simulink model "dq_current_controller_discrete"  (R2025b)
settings: Solver=FixedStepDiscrete  FixedStep=control.currentLoopPeriod_s
undefined symbols (not defined in the file): control, DiscIntNeverNeededParam, motor
settings Model: Creator=semih  LastModifiedBy=Semih
settings SFSimCC: SimGPUStackLimitPerThread=51200  SimGPUMallocThreshold=200
settings RTWCC: GPUStackLimitPerThread=51200  GPUMallocThreshold=200
settings GRTTargetCC: CombineOutputUpdateFcns=off

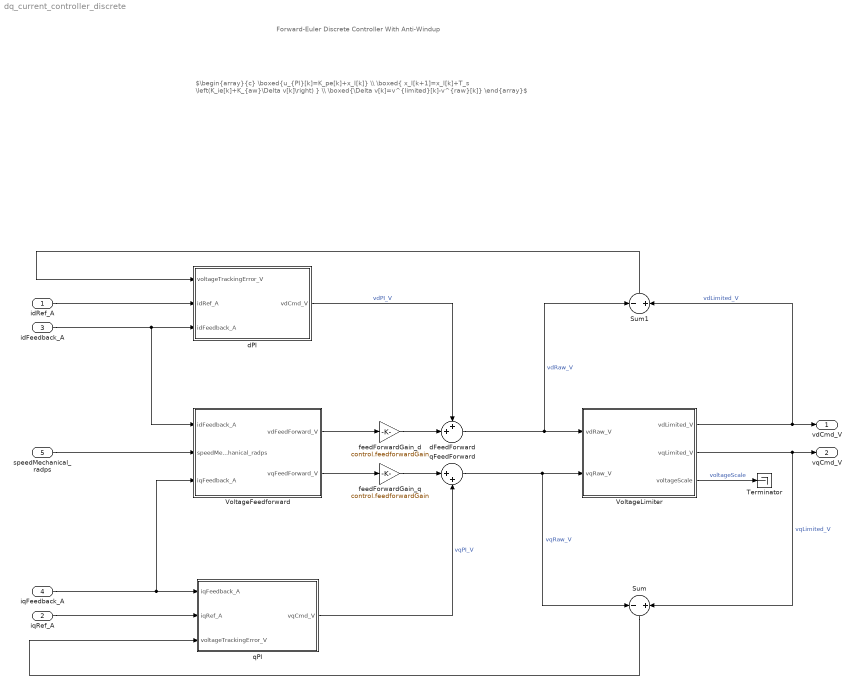
== system dq_current_controller_discrete ==
  note: $\begin{array}{c} \boxed{u_{PI}[k]=K_pe[k]+x_I[k]} \\ \boxed{ x_I[k+1]=x_I[k]+T_s \left(K_ie[k]+K_{aw}\Delta v[k]\right) } \\ \boxed{\Delta v[k]=v^{limited}[k]-v^{raw}[k]} \end{array}$
  note: Forward-Euler Discrete Controller
      | With Anti-Windup
  idRef_A : Inport
  iqRef_A : Inport  Port=2
  idFeedback_A : Inport  Port=3
  iqFeedback_A : Inport  Port=4
  speedMechanical_radps : Inport  Port=5
  Sum : Sum  Inputs=-+
  Sum1 : Sum  Inputs=-+
  Terminator : Terminator
  VoltageFeedforward : Subsystem
  VoltageLimiter : Subsystem
  dFeedForward : Sum  Inputs=++|
  dPI : Subsystem
  feedForwardGain_d : Gain  Gain=control.feedforwardGain
  feedForwardGain_q : Gain  Gain=control.feedforwardGain
  qFeedForward : Sum  Inputs=|++
  qPI : Subsystem
  vdCmd_V : Outport
  vqCmd_V : Outport  Port=2
  wires:
  dPI/1(vdCmd_V) -> dFeedForward/1  "vdPI_V"
  qPI/1(vqCmd_V) -> qFeedForward/2  "vqPI_V"
  VoltageFeedforward/2(vqFeedForward_V) -> feedForwardGain_q/1
  VoltageFeedforward/1(vdFeedForward_V) -> feedForwardGain_d/1
  feedForwardGain_q/1 -> qFeedForward/1
  feedForwardGain_d/1 -> dFeedForward/2
  idRef_A/1 -> dPI/2(idRef_A)
  idFeedback_A/1 -> VoltageFeedforward/1(idFeedback_A), dPI/3(idFeedback_A)
  speedMechanical_radps/1 -> VoltageFeedforward/2(speedMechanical_radps)
  iqFeedback_A/1 -> qPI/1(iqFeedback_A), VoltageFeedforward/3(iqFeedback_A)
  dFeedForward/1 -> Sum1/1, VoltageLimiter/1(vdRaw_V)  "vdRaw_V"
  qFeedForward/1 -> Sum/1, VoltageLimiter/2(vqRaw_V)  "vqRaw_V"
  VoltageLimiter/1(vdLimited_V) -> Sum1/2, vdCmd_V/1  "vdLimited_V"
  VoltageLimiter/2(vqLimited_V) -> Sum/2, vqCmd_V/1  "vqLimited_V"
  VoltageLimiter/3(voltageScale) -> Terminator/1  "voltageScale"
  Sum1/1 -> dPI/1(voltageTrackingError_V)
  Sum/1 -> qPI/3(voltageTrackingError_V)
  iqRef_A/1 -> qPI/2(iqRef_A)

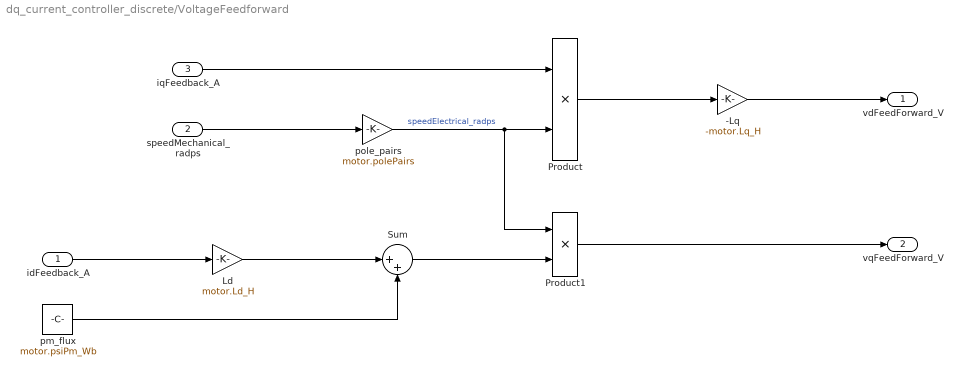
== system dq_current_controller_discrete/VoltageFeedforward ==
  idFeedback_A : Inport
  speedMechanical_radps : Inport  Port=2
  iqFeedback_A : Inport  Port=3
  -Lq : Gain  Gain=-motor.Lq_H
  Ld : Gain  Gain=motor.Ld_H
  Product : Product
  Product1 : Product
  Sum : Sum  Inputs=|++
  pm_flux : Constant  Value=motor.psiPm_Wb
  pole_pairs : Gain  Gain=motor.polePairs
  vdFeedForward_V : Outport
  vqFeedForward_V : Outport  Port=2
  wires:
  speedMechanical_radps/1 -> pole_pairs/1
  pole_pairs/1 -> Product1/1, Product/2  "speedElectrical_radps"
  iqFeedback_A/1 -> Product/1
  Product/1 -> -Lq/1
  -Lq/1 -> vdFeedForward_V/1
  idFeedback_A/1 -> Ld/1
  pm_flux/1 -> Sum/2
  Ld/1 -> Sum/1
  Sum/1 -> Product1/2
  Product1/1 -> vqFeedForward_V/1

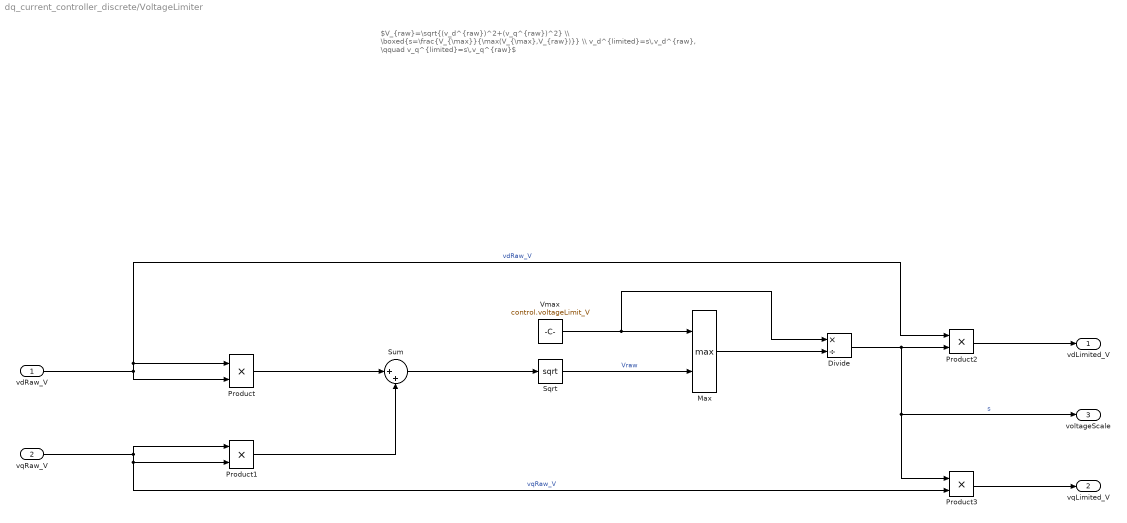
== system dq_current_controller_discrete/VoltageLimiter ==
  note: $V_{raw}=\sqrt{(v_d^{raw})^2+(v_q^{raw})^2} \\ \boxed{s=\frac{V_{\max}}{\max(V_{\max},V_{raw})}} \\ v_d^{limited}=s\,v_d^{raw}, \qquad v_q^{limited}=s\,v_q^{raw}$
  vdRaw_V : Inport
  vqRaw_V : Inport  Port=2
  Divide : Product  Inputs=*/
  Max : MinMax  Function=max  Inputs=2
  Product{,1..3} (4 alike) : Product
  Sqrt : Sqrt
  Sum : Sum  Inputs=|++
  Vmax : Constant  Value=control.voltageLimit_V
  vdLimited_V : Outport
  vqLimited_V : Outport  Port=2
  voltageScale : Outport  Port=3
  wires:
  vdRaw_V/1 -> Product2/1, Product/1, Product/2  "vdRaw_V"
  vqRaw_V/1 -> Product1/2, Product3/2, Product1/1  "vqRaw_V"
  Product/1 -> Sum/1
  Product1/1 -> Sum/2
  Sum/1 -> Sqrt/1
  Sqrt/1 -> Max/2  "Vraw"
  Vmax/1 -> Divide/1, Max/1
  Max/1 -> Divide/2
  Divide/1 -> voltageScale/1, Product3/1, Product2/2  "s"
  Product2/1 -> vdLimited_V/1
  Product3/1 -> vqLimited_V/1

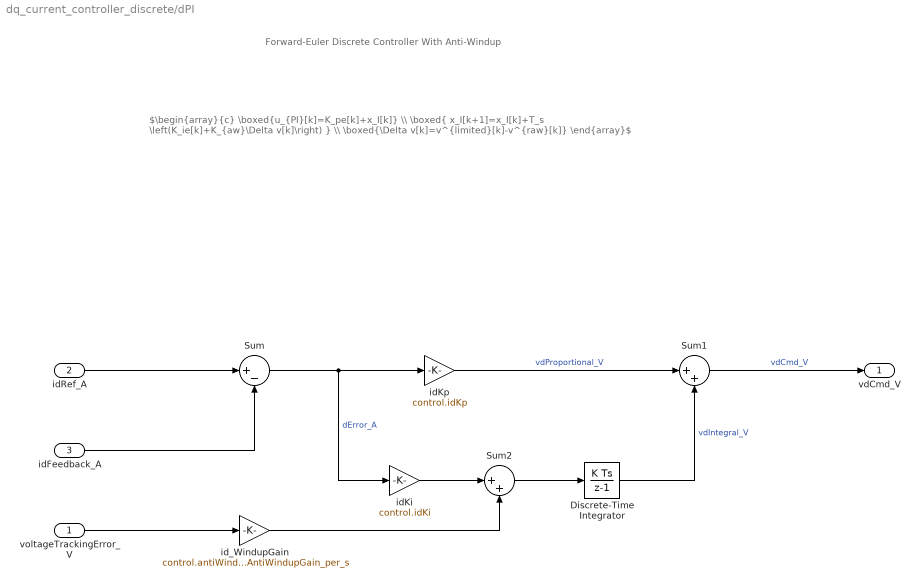
== system dq_current_controller_discrete/dPI ==
  note: Forward-Euler Discrete Controller
      | With Anti-Windup
  note: $\begin{array}{c} \boxed{u_{PI}[k]=K_pe[k]+x_I[k]} \\ \boxed{ x_I[k+1]=x_I[k]+T_s \left(K_ie[k]+K_{aw}\Delta v[k]\right) } \\ \boxed{\Delta v[k]=v^{limited}[k]-v^{raw}[k]} \end{array}$
  voltageTrackingError_V : Inport
  idRef_A : Inport  Port=2
  idFeedback_A : Inport  Port=3
  Discrete-Time Integrator : DiscreteIntegrator  SampleTime=control.currentLoopPeriod_s  ICPrevOutput=DiscIntNeverNeededParam  ICPrevScaledInput=DiscIntNeverNeededParam
  Sum : Sum  Inputs=|+-
  Sum1 : Sum  Inputs=|++
  Sum2 : Sum  Inputs=|++
  idKi : Gain  Gain=control.idKi
  idKp : Gain  Gain=control.idKp
  id_WindupGain : Gain  Gain=control.antiWindupEnable * control.idAntiWindupGain_per_s
  vdCmd_V : Outport
  wires:
  idFeedback_A/1 -> Sum/2
  idKp/1 -> Sum1/1  "vdProportional_V"
  Discrete-Time Integrator/1 -> Sum1/2  "vdIntegral_V"
  idRef_A/1 -> Sum/1
  Sum1/1 -> vdCmd_V/1  "vdCmd_V"
  Sum/1 -> idKp/1, idKi/1  "dError_A"
  idKi/1 -> Sum2/1
  Sum2/1 -> Discrete-Time Integrator/1
  voltageTrackingError_V/1 -> id_WindupGain/1
  id_WindupGain/1 -> Sum2/2

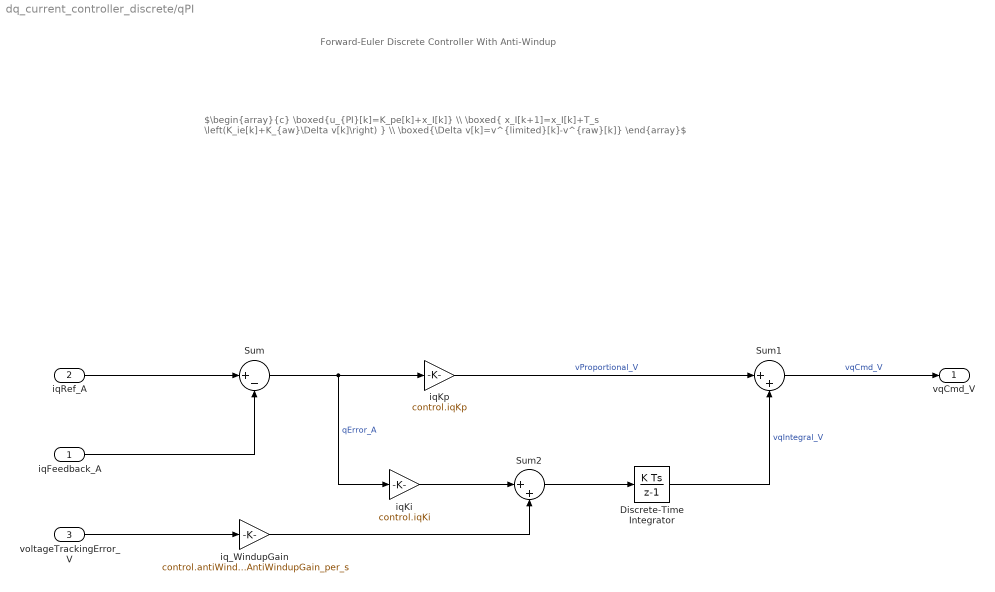
== system dq_current_controller_discrete/qPI ==
  note: $\begin{array}{c} \boxed{u_{PI}[k]=K_pe[k]+x_I[k]} \\ \boxed{ x_I[k+1]=x_I[k]+T_s \left(K_ie[k]+K_{aw}\Delta v[k]\right) } \\ \boxed{\Delta v[k]=v^{limited}[k]-v^{raw}[k]} \end{array}$
  note: Forward-Euler Discrete Controller
      | With Anti-Windup
  iqFeedback_A : Inport
  iqRef_A : Inport  Port=2
  voltageTrackingError_V : Inport  Port=3
  Discrete-Time Integrator : DiscreteIntegrator  SampleTime=control.currentLoopPeriod_s  ICPrevOutput=DiscIntNeverNeededParam  ICPrevScaledInput=DiscIntNeverNeededParam
  Sum : Sum  Inputs=|+-
  Sum1 : Sum  Inputs=|++
  Sum2 : Sum  Inputs=|++
  iqKi : Gain  Gain=control.iqKi
  iqKp : Gain  Gain=control.iqKp
  iq_WindupGain : Gain  Gain=control.antiWindupEnable * control.iqAntiWindupGain_per_s
  vqCmd_V : Outport
  wires:
  Discrete-Time Integrator/1 -> Sum1/2  "vqIntegral_V"
  iqRef_A/1 -> Sum/1
  Sum1/1 -> vqCmd_V/1  "vqCmd_V"
  iqFeedback_A/1 -> Sum/2
  Sum/1 -> iqKp/1, iqKi/1  "qError_A"
  iqKp/1 -> Sum1/1  "vProportional_V"
  iqKi/1 -> Sum2/1
  voltageTrackingError_V/1 -> iq_WindupGain/1
  iq_WindupGain/1 -> Sum2/2
  Sum2/1 -> Discrete-Time Integrator/1
